simulink model "Voltage_Control"  (R2026b)
undefined symbols (not defined in the file): ctrlOut, isAtSetpoint, rampedSetpoint, VoltageControl_max, VoltageControl_min, VoltageControl_ts
libraries: simulink x2, slpidlib x1, sl_discontinuities x1
settings Model: Creator=BenjaminRupp  LastModifiedBy=BenjaminRupp

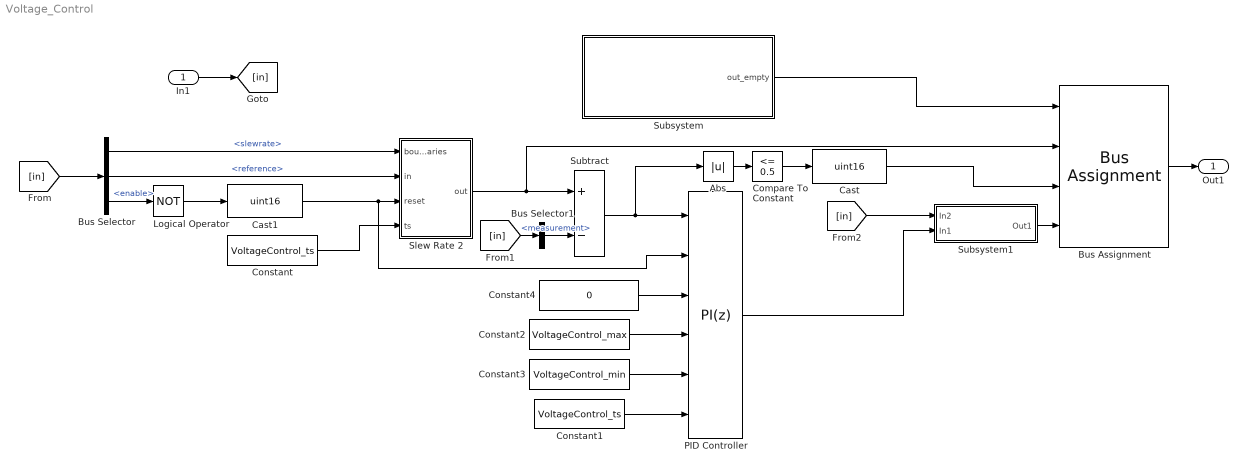
== system Voltage_Control ==
  In1 : Inport  OutDataTypeStr=Bus: VoltageControl_in
  Abs : Abs  SaturateOnIntegerOverflow=off
  Bus Assignment : BusAssignment  AssignedSignals=rampedSetpoint,isAtSetpoint,ctrlOut
  Bus Selector : BusSelector  OutputSignals=slewrate,reference,enable
  Bus Selector1 : BusSelector  OutputSignals=measurement
  Cast : DataTypeConversion  OutDataTypeStr=uint16  SaturateOnIntegerOverflow=off  RndMeth=Floor
  Cast1 : DataTypeConversion  OutDataTypeStr=uint16  SaturateOnIntegerOverflow=off  RndMeth=Floor
  Compare To Constant : simulink/Logic and Bit Operations/Compare To Constant  relop=<=  const=0.5  OutDataTypeStr=uint8
  Constant : Constant  Value=VoltageControl_ts  OutDataTypeStr=single
  Constant1 : Constant  Value=VoltageControl_ts  OutDataTypeStr=single  SampleTime=-1
  Constant2 : Constant  Value=VoltageControl_max  OutDataTypeStr=single  SampleTime=-1
  Constant3 : Constant  Value=VoltageControl_min  OutDataTypeStr=single  SampleTime=-1
  Constant4 : Constant  Value=0  OutDataTypeStr=single  SampleTime=-1
  Logical Operator : Logic  Operator=NOT  AllPortsSameDT=off  OutDataTypeStr=boolean
  PID Controller : slpidlib/PID Controller  Controller=PI  Form=Parallel  TimeDomain=Discrete-time  UseExternalTs=on  SampleTime=-1  IntegratorMethod=Forward Euler  FilterMethod=Forward Euler  ControllerParametersSource=internal  P=0.01  I=1  UseKiTs=off  D=0  UseExternalDerivativeSource=off  N=100  UseFilter=on  TunerSelectOption=Transfer Function Based (PID Tuner App)  InitialConditionSource=external  InitialConditionForIntegrator=0  InitialConditionForFilter=0  DifferentiatorICPrevScaledInput=0  ExternalReset=level  TrackingMode=off  Kt=1  LimitOutput=on  SatLimitsSource=external  UpperSaturationLimit=inf  LowerSaturationLimit=-inf  LinearizeAsGain=on  AntiWindupMode=clamping  Kb=1  LimitIntegrator=off  UpperIntegratorSaturationLimit=inf  LowerIntegratorSaturationLimit=-inf  POutMin=[]  POutMax=[]  IOutMin=[]  IOutMax=[]  DOutMin=[]  DOutMax=[]  NOutMin=[]  NOutMax=[]  SumOutMin=[]  SumOutMax=[]  SaturationOutMin=[]  SaturationOutMax=[]  PParamMin=[]  PParamMax=[]  IParamMin=[]  IParamMax=[]  DParamMin=[]  DParamMax=[]  NParamMin=[]  NParamMax=[]  KbParamMin=[]  KbParamMax=[]  KtParamMin=[]  KtParamMax=[]  KbOutMin=[]  KbOutMax=[]  KtOutMin=[]  KtOutMax=[]  IntegratorOutMin=[]  IntegratorOutMax=[]  FilterOutMin=[]  FilterOutMax=[]  SumI1OutMin=[]  SumI1OutMax=[]  SumI2OutMin=[]  SumI2OutMax=[]  SumI3OutMin=[]  SumI3OutMax=[]  SumI4OutMin=[]  SumI4OutMax=[]  SumDOutMin=[]  SumDOutMax=[]  DifferentiatorOutMin=[]  DifferentiatorOutMax=[]  FilterDiffOutCoefMin=[]  FilterDiffOutCoefMax=[]  ReciprocalOutMin=[]  ReciprocalOutMax=[]  SumDenOutMin=[]  SumDenOutMax=[]  SumNumOutMin=[]  SumNumOutMax=[]  DivideOutMin=[]  DivideOutMax=[]  UdiffTsProdOutMin=[]  UdiffTsProdOutMax=[]  NTsProdOutMin=[]  NTsProdOutMax=[]  UintegralTsProdOutMin=[]  UintegralTsProdOutMax=[]  UngainTsProdOutMin=[]  UngainTsProdOutMax=[]  ClampingZeroOutDataTypeStr=Inherit: Inherit via back propagation  ClampingZeroOutMin=[]  ClampingZeroOutMax=[]  FilterDenConstantOutDataTypeStr=Inherit: Inherit via back propagation  FilterDenConstantOutMin=[]  FilterDenConstantOutMax=[]  PCopyOutDataTypeStr=Inherit: Inherit via back propagation  PCopyOutMin=[]  PCopyOutMax=[]  NCopyOutDataTypeStr=Inherit: Inherit via back propagation  NCopyOutMin=[]  NCopyOutMax=[]  IntegratorContinuousStateAttributes=''  IntegratorStateMustResolveToSignalObject=off  IntegratorRTWStateStorageClass=Auto  FilterContinuousStateAttributes=''  FilterStateMustResolveToSignalObject=off  FilterRTWStateStorageClass=Auto  ParallelPVariant=InternalParameters  IdealPVariant=Disabled  IVariant=InternalParameters  DVariant=Disabled  IntegratorVariant=Discrete  SatVariant=External  AWVariant=DiscClampingParallel  PCopyVariant=Disabled  TRVariant=Disabled  FdbkBlocksVariant=Forward  IdealPFdbkVariant=Disabled  SatFdbkVariant=Disabled  DerivativeFilterVariant=Disabled  NVariant=Disabled  NCopyVariant=Disabled_SignalSpec  FilterICVariant=Disabled  IntegratorICVariant=ExternalICs  ExternalResetVariant=ExternalReset  TRSumVariant=Passthrough  SumFdbkVariant=Disabled  SumVariant=Sum_PI  TsampFilterVariant=InternalTs  TsampNgainVariant=Passthrough  TsampIntegralVariant=ExternalTs  ExternalSaturationOutDataTypeStr=Inherit: Same as second input  DerivativeSourceVariant=Disabled  PreIntVariant=InternalPreInt
  Slew Rate 2 : Subsystem  mask{IcPosSlewRate=100e3, IcNegSlewRate=-100e3}
      mask prompts: IcPosSlewRate "Initial Condition Positive Slew Rate"; IcNegSlewRate "Initial Condition Negative Slew Rate"
  Subsystem : Subsystem
  Subsystem1 : Subsystem
  Subtract : Sum  Inputs=+-
  Out1 : Outport  OutDataTypeStr=Bus: VoltageControl_out
  wires:
  Constant1/1 -> PID Controller/6
  Constant4/1 -> PID Controller/3
  In1/1 -> [in]
  Bus Selector1/1 -> Subtract/2  "<measurement>"
  Subsystem/1(out_empty) -> Bus Assignment/1
  Bus Selector/1 -> Slew Rate 2/1(boundaries)  "<slewrate>"
  [in] -> Bus Selector1/1
  Logical Operator/1 -> Cast1/1
  Abs/1 -> Compare To Constant/1
  Cast1/1 -> PID Controller/2, Slew Rate 2/3(reset)
  Cast/1 -> Bus Assignment/3
  Bus Assignment/1 -> Out1/1
  Bus Selector/3 -> Logical Operator/1  "<enable>"
  Subtract/1 -> Abs/1, PID Controller/1
  Constant2/1 -> PID Controller/4
  Constant/1 -> Slew Rate 2/4(ts)
  Constant3/1 -> PID Controller/5
  Slew Rate 2/1(out) -> Bus Assignment/2, Subtract/1
  Compare To Constant/1 -> Cast/1
  [in] -> Bus Selector/1
  Bus Selector/2 -> Slew Rate 2/2(in)  "<reference>"
  PID Controller/1 -> Subsystem1/2(In1)
  [in] -> Subsystem1/1(In2)
  Subsystem1/1(Out1) -> Bus Assignment/4

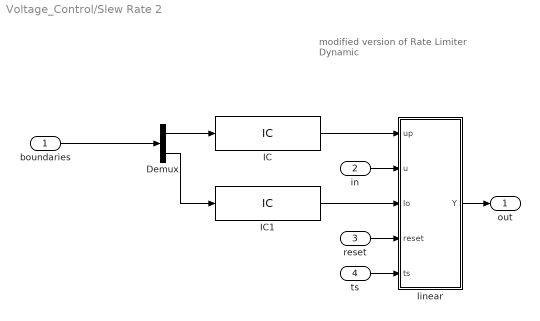
== system Voltage_Control/Slew Rate 2 ==
  note: modified version of Rate Limiter
      | Dynamic
  boundaries : Inport
  in : Inport  Port=2
  reset : Inport  Port=3
  ts : Inport  Port=4
  Demux : Demux  Outputs=2
  IC : InitialCondition  Value=IcPosSlewRate
  IC1 : InitialCondition  Value=IcNegSlewRate
  linear : Subsystem
  out : Outport
  wires:
  reset/1 -> linear/4(reset)
  IC1/1 -> linear/3(lo)
  IC/1 -> linear/1(up)
  linear/1(Y) -> out/1
  in/1 -> linear/2(u)
  Demux/2 -> IC1/1
  Demux/1 -> IC/1
  boundaries/1 -> Demux/1
  ts/1 -> linear/5(ts)

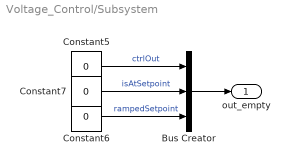
== system Voltage_Control/Subsystem ==
  Bus Creator : BusCreator  Inputs=3  OutDataTypeStr=Bus: VoltageControl_out
  Constant5 : Constant  Value=0  OutDataTypeStr=single  SampleTime=-1
  Constant6 : Constant  Value=0  OutDataTypeStr=single  SampleTime=-1
  Constant7 : Constant  Value=0  OutDataTypeStr=uint16  SampleTime=-1
  out_empty : Outport
  wires:
  Bus Creator/1 -> out_empty/1
  Constant5/1 -> Bus Creator/1  "ctrlOut"
  Constant6/1 -> Bus Creator/3  "rampedSetpoint"
  Constant7/1 -> Bus Creator/2  "isAtSetpoint"

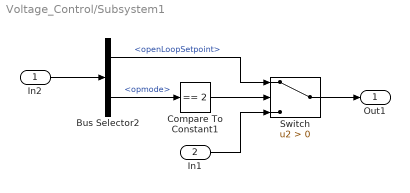
== system Voltage_Control/Subsystem1 ==
  In2 : Inport
  In1 : Inport  Port=2
  Bus Selector2 : BusSelector  OutputSignals=openLoopSetpoint,opmode
  Compare To Constant1 : simulink/Logic and Bit Operations/Compare To Constant  relop===  const=2  OutDataTypeStr=boolean
  Switch : Switch  Criteria=u2 > Threshold  SaturateOnIntegerOverflow=off  InputSameDT=off
  Out1 : Outport
  wires:
  Bus Selector2/2 -> Compare To Constant1/1  "<opmode>"
  In2/1 -> Bus Selector2/1
  Compare To Constant1/1 -> Switch/2
  Bus Selector2/1 -> Switch/1  "<openLoopSetpoint>"
  Switch/1 -> Out1/1
  In1/1 -> Switch/3

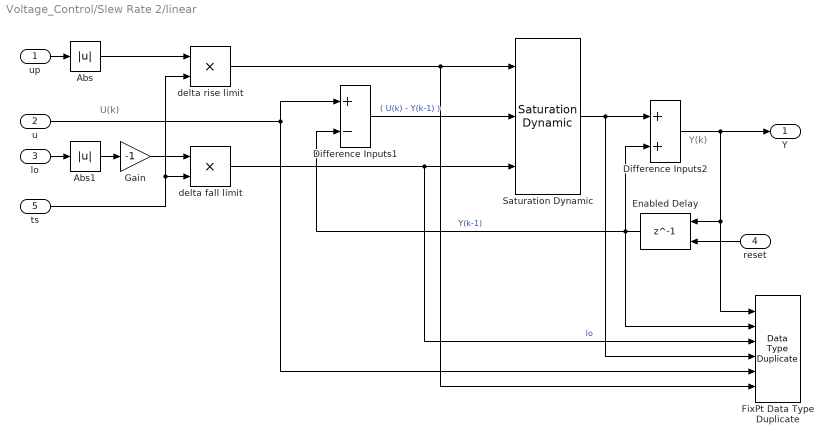
== system Voltage_Control/Slew Rate 2/linear ==
  note: U(k)
  note: Y(k)
  up : Inport
  u : Inport  Port=2
  lo : Inport  Port=3
  reset : Inport  Port=4
  ts : Inport  Port=5
  Abs : Abs  ZeroCross=off  SaturateOnIntegerOverflow=off
  Abs1 : Abs  ZeroCross=off  SaturateOnIntegerOverflow=off
  Difference Inputs1 : Sum  Description=Add in CPU  DisableCoverage=on  Inputs=+-  OutDataTypeStr=Inherit: Inherit via back propagation
  Difference Inputs2 : Sum  Description=Add in CPU  OutDataTypeStr=Inherit: Inherit via back propagation
  Enabled Delay : Delay  DelayLength=1  ExternalReset=Level
      settings: InputPortMap=u0,r5
  FixPt Data Type Duplicate : DataTypeDuplicate  DisableCoverage=on  NumInputPorts=6
  Gain : Gain  Gain=-1
  Saturation Dynamic : sl_discontinuities/Saturation Dynamic  OutMin=[]  OutMax=[]  OutDataTypeStr=Inherit: Same as second input  OutDataType=fixdt(1, 16)  OutScaling=2^-10  DoSatur=off
  delta fall limit : Product  DisableCoverage=on  Inputs=**  OutDataTypeStr=Inherit: Inherit via back propagation  SaturateOnIntegerOverflow=on
  delta rise limit : Product  DisableCoverage=on  Inputs=**  OutDataTypeStr=Inherit: Inherit via back propagation  SaturateOnIntegerOverflow=on
  Y : Outport
  wires:
  reset/1 -> Enabled Delay/2
  delta fall limit/1 -> FixPt Data Type Duplicate/3, Saturation Dynamic/3  "lo"
  Saturation Dynamic/1 -> FixPt Data Type Duplicate/4, Difference Inputs2/1
  Difference Inputs1/1 -> Saturation Dynamic/2  "( U(k) - Y(k-1) )"
  u/1 -> FixPt Data Type Duplicate/5, Difference Inputs1/1
  ts/1 -> delta fall limit/2, delta rise limit/2
  up/1 -> Abs/1
  delta rise limit/1 -> FixPt Data Type Duplicate/6, Saturation Dynamic/1
  Enabled Delay/1 -> FixPt Data Type Duplicate/2, Difference Inputs2/2, Difference Inputs1/2  "Y(k-1)"
  Difference Inputs2/1 -> FixPt Data Type Duplicate/1, Enabled Delay/1, Y/1
  Abs/1 -> delta rise limit/1
  lo/1 -> Abs1/1
  Abs1/1 -> Gain/1
  Gain/1 -> delta fall limit/1
